simulink model "ASM_Traffic_new"  (R2024a)
settings: Solver=ode1  StartTime=SIM.tstart.v  StopTime=SIM.tend.v  FixedStep=SIM.StepSize.v  RelTol=1e-3
PostLoadFcn:
  | if any(exist('dsrtsu_mdlpostloadfcn', 'file') ~= 0), dsrtsu_mdlpostloadfcn('Execute', bdroot); end
  | try, asm_mdl_postloadfcn(bdroot, 'UpdateModel', 3600); catch, disp(lasterr); end,
InitFcn:
  | , if any(exist('rtifpga_mdlclblib', 'file') ~= 0), rtifpga_mdlclblib('Init', bdroot); end,
  | , if any(exist('dsmpb_private', 'file') ~= 0), dsmpb_private('dsmpb_mdlclblib', 'Init', bdroot); end,
undefined symbols (not defined in the file): _to_, a0b2, ASM_BrakeHydraulics_DemoSystems, ASM_VehicleDynamics_DemoSystems, b98103fe8ad365046cd0, BrakeCircuit, CPT, Crankshaft, DiscIntNeverNeededParam, dsmsi, FinalDriveAssembly, MDL, ModeSignals, Pos_BrakePedal_Maneuver, rad, RefSignals, s_to_rpm, SIM, SoftECU, Suspension, Tire, Transmission
libraries: ASM_Traffic_lib x135, simulink x100, ASM_Utils_lib x77, ASM_VehicleDynamics_lib x70, ASM_Environment_lib x22, dsmpblib x20, dsmsilib x15, MDLD_Utils_lib x10, ASM_BrakeHydraulics_lib x3
(part 52 of 63)

== system ASM_Traffic_new/Environment/Traffic/UserInterface/PAR_Plant/Fellow_Doors/Fellow26_Doors ==
  Bus Creator1 : BusCreator  Inputs=7
  SW_DoorFL[0Closed_1Open] : Constant  Value=0
  SW_DoorFR[0Closed_1Open] : Constant  Value=0
  SW_DoorRL[0Closed_1Open] : Constant  Value=0
  SW_DoorRR[0Closed_1Open] : Constant  Value=0
  SW_Hood[0Closed_1Open] : Constant  Value=0
  SW_ManualControl_Doors[1Scheduler|2Manual] : Constant
  SW_Trunk[0Closed_1Open] : Constant  Value=0
  Out1 : Outport  VectorParamsAs1DForOutWhenUnconnected=off
  wires:
  Bus Creator1/1 -> Out1/1
  SW_ManualControl_Doors[1Scheduler|2Manual]/1 -> Bus Creator1/1  "SW_ManualControl_Doors[1Scheduler|2Manual]"
  SW_DoorFL[0Closed_1Open]/1 -> Bus Creator1/2  "SW_DoorFL[0Closed_1Open]"
  SW_DoorFR[0Closed_1Open]/1 -> Bus Creator1/3  "SW_DoorFR[0Closed_1Open]"
  SW_DoorRL[0Closed_1Open]/1 -> Bus Creator1/4  "SW_DoorRL[0Closed_1Open]"
  SW_DoorRR[0Closed_1Open]/1 -> Bus Creator1/5  "SW_DoorRR[0Closed_1Open]"
  SW_Hood[0Closed_1Open]/1 -> Bus Creator1/6  "SW_Hood[0Closed_1Open]"
  SW_Trunk[0Closed_1Open]/1 -> Bus Creator1/7  "SW_Trunk[0Closed_1Open]"

== system ASM_Traffic_new/Environment/Traffic/UserInterface/PAR_Plant/Fellow_Doors/Fellow27_Doors ==
  Bus Creator1 : BusCreator  Inputs=7
  SW_DoorFL[0Closed_1Open] : Constant  Value=0
  SW_DoorFR[0Closed_1Open] : Constant  Value=0
  SW_DoorRL[0Closed_1Open] : Constant  Value=0
  SW_DoorRR[0Closed_1Open] : Constant  Value=0
  SW_Hood[0Closed_1Open] : Constant  Value=0
  SW_ManualControl_Doors[1Scheduler|2Manual] : Constant
  SW_Trunk[0Closed_1Open] : Constant  Value=0
  Out1 : Outport  VectorParamsAs1DForOutWhenUnconnected=off
  wires:
  Bus Creator1/1 -> Out1/1
  SW_ManualControl_Doors[1Scheduler|2Manual]/1 -> Bus Creator1/1  "SW_ManualControl_Doors[1Scheduler|2Manual]"
  SW_DoorFL[0Closed_1Open]/1 -> Bus Creator1/2  "SW_DoorFL[0Closed_1Open]"
  SW_DoorFR[0Closed_1Open]/1 -> Bus Creator1/3  "SW_DoorFR[0Closed_1Open]"
  SW_DoorRL[0Closed_1Open]/1 -> Bus Creator1/4  "SW_DoorRL[0Closed_1Open]"
  SW_DoorRR[0Closed_1Open]/1 -> Bus Creator1/5  "SW_DoorRR[0Closed_1Open]"
  SW_Hood[0Closed_1Open]/1 -> Bus Creator1/6  "SW_Hood[0Closed_1Open]"
  SW_Trunk[0Closed_1Open]/1 -> Bus Creator1/7  "SW_Trunk[0Closed_1Open]"

== system ASM_Traffic_new/Environment/Traffic/UserInterface/PAR_Plant/Fellow_Doors/Fellow28_Doors ==
  Bus Creator1 : BusCreator  Inputs=7
  SW_DoorFL[0Closed_1Open] : Constant  Value=0
  SW_DoorFR[0Closed_1Open] : Constant  Value=0
  SW_DoorRL[0Closed_1Open] : Constant  Value=0
  SW_DoorRR[0Closed_1Open] : Constant  Value=0
  SW_Hood[0Closed_1Open] : Constant  Value=0
  SW_ManualControl_Doors[1Scheduler|2Manual] : Constant
  SW_Trunk[0Closed_1Open] : Constant  Value=0
  Out1 : Outport  VectorParamsAs1DForOutWhenUnconnected=off
  wires:
  Bus Creator1/1 -> Out1/1
  SW_ManualControl_Doors[1Scheduler|2Manual]/1 -> Bus Creator1/1  "SW_ManualControl_Doors[1Scheduler|2Manual]"
  SW_DoorFL[0Closed_1Open]/1 -> Bus Creator1/2  "SW_DoorFL[0Closed_1Open]"
  SW_DoorFR[0Closed_1Open]/1 -> Bus Creator1/3  "SW_DoorFR[0Closed_1Open]"
  SW_DoorRL[0Closed_1Open]/1 -> Bus Creator1/4  "SW_DoorRL[0Closed_1Open]"
  SW_DoorRR[0Closed_1Open]/1 -> Bus Creator1/5  "SW_DoorRR[0Closed_1Open]"
  SW_Hood[0Closed_1Open]/1 -> Bus Creator1/6  "SW_Hood[0Closed_1Open]"
  SW_Trunk[0Closed_1Open]/1 -> Bus Creator1/7  "SW_Trunk[0Closed_1Open]"

== system ASM_Traffic_new/Environment/Traffic/UserInterface/PAR_Plant/Fellow_Doors/Fellow29_Doors ==
  Bus Creator1 : BusCreator  Inputs=7
  SW_DoorFL[0Closed_1Open] : Constant  Value=0
  SW_DoorFR[0Closed_1Open] : Constant  Value=0
  SW_DoorRL[0Closed_1Open] : Constant  Value=0
  SW_DoorRR[0Closed_1Open] : Constant  Value=0
  SW_Hood[0Closed_1Open] : Constant  Value=0
  SW_ManualControl_Doors[1Scheduler|2Manual] : Constant
  SW_Trunk[0Closed_1Open] : Constant  Value=0
  Out1 : Outport  VectorParamsAs1DForOutWhenUnconnected=off
  wires:
  Bus Creator1/1 -> Out1/1
  SW_ManualControl_Doors[1Scheduler|2Manual]/1 -> Bus Creator1/1  "SW_ManualControl_Doors[1Scheduler|2Manual]"
  SW_DoorFL[0Closed_1Open]/1 -> Bus Creator1/2  "SW_DoorFL[0Closed_1Open]"
  SW_DoorFR[0Closed_1Open]/1 -> Bus Creator1/3  "SW_DoorFR[0Closed_1Open]"
  SW_DoorRL[0Closed_1Open]/1 -> Bus Creator1/4  "SW_DoorRL[0Closed_1Open]"
  SW_DoorRR[0Closed_1Open]/1 -> Bus Creator1/5  "SW_DoorRR[0Closed_1Open]"
  SW_Hood[0Closed_1Open]/1 -> Bus Creator1/6  "SW_Hood[0Closed_1Open]"
  SW_Trunk[0Closed_1Open]/1 -> Bus Creator1/7  "SW_Trunk[0Closed_1Open]"

== system ASM_Traffic_new/Environment/Traffic/UserInterface/PAR_Plant/Fellow_Doors/Fellow2_Doors ==
  Bus Creator1 : BusCreator  Inputs=7
  SW_DoorFL[0Closed_1Open] : Constant  Value=0
  SW_DoorFR[0Closed_1Open] : Constant  Value=0
  SW_DoorRL[0Closed_1Open] : Constant  Value=0
  SW_DoorRR[0Closed_1Open] : Constant  Value=0
  SW_Hood[0Closed_1Open] : Constant  Value=0
  SW_ManualControl_Doors[1Scheduler|2Manual] : Constant
  SW_Trunk[0Closed_1Open] : Constant  Value=0
  Out1 : Outport  VectorParamsAs1DForOutWhenUnconnected=off
  wires:
  Bus Creator1/1 -> Out1/1
  SW_ManualControl_Doors[1Scheduler|2Manual]/1 -> Bus Creator1/1  "SW_ManualControl_Doors[1Scheduler|2Manual]"
  SW_DoorFL[0Closed_1Open]/1 -> Bus Creator1/2  "SW_DoorFL[0Closed_1Open]"
  SW_DoorFR[0Closed_1Open]/1 -> Bus Creator1/3  "SW_DoorFR[0Closed_1Open]"
  SW_DoorRL[0Closed_1Open]/1 -> Bus Creator1/4  "SW_DoorRL[0Closed_1Open]"
  SW_DoorRR[0Closed_1Open]/1 -> Bus Creator1/5  "SW_DoorRR[0Closed_1Open]"
  SW_Hood[0Closed_1Open]/1 -> Bus Creator1/6  "SW_Hood[0Closed_1Open]"
  SW_Trunk[0Closed_1Open]/1 -> Bus Creator1/7  "SW_Trunk[0Closed_1Open]"

== system ASM_Traffic_new/Environment/Traffic/UserInterface/PAR_Plant/Fellow_Doors/Fellow30_Doors ==
  Bus Creator1 : BusCreator  Inputs=7
  SW_DoorFL[0Closed_1Open] : Constant  Value=0
  SW_DoorFR[0Closed_1Open] : Constant  Value=0
  SW_DoorRL[0Closed_1Open] : Constant  Value=0
  SW_DoorRR[0Closed_1Open] : Constant  Value=0
  SW_Hood[0Closed_1Open] : Constant  Value=0
  SW_ManualControl_Doors[1Scheduler|2Manual] : Constant
  SW_Trunk[0Closed_1Open] : Constant  Value=0
  Out1 : Outport  VectorParamsAs1DForOutWhenUnconnected=off
  wires:
  Bus Creator1/1 -> Out1/1
  SW_ManualControl_Doors[1Scheduler|2Manual]/1 -> Bus Creator1/1  "SW_ManualControl_Doors[1Scheduler|2Manual]"
  SW_DoorFL[0Closed_1Open]/1 -> Bus Creator1/2  "SW_DoorFL[0Closed_1Open]"
  SW_DoorFR[0Closed_1Open]/1 -> Bus Creator1/3  "SW_DoorFR[0Closed_1Open]"
  SW_DoorRL[0Closed_1Open]/1 -> Bus Creator1/4  "SW_DoorRL[0Closed_1Open]"
  SW_DoorRR[0Closed_1Open]/1 -> Bus Creator1/5  "SW_DoorRR[0Closed_1Open]"
  SW_Hood[0Closed_1Open]/1 -> Bus Creator1/6  "SW_Hood[0Closed_1Open]"
  SW_Trunk[0Closed_1Open]/1 -> Bus Creator1/7  "SW_Trunk[0Closed_1Open]"

== system ASM_Traffic_new/Environment/Traffic/UserInterface/PAR_Plant/Fellow_Doors/Fellow3_Doors ==
  Bus Creator1 : BusCreator  Inputs=7
  SW_DoorFL[0Closed_1Open] : Constant  Value=0
  SW_DoorFR[0Closed_1Open] : Constant  Value=0
  SW_DoorRL[0Closed_1Open] : Constant  Value=0
  SW_DoorRR[0Closed_1Open] : Constant  Value=0
  SW_Hood[0Closed_1Open] : Constant  Value=0
  SW_ManualControl_Doors[1Scheduler|2Manual] : Constant
  SW_Trunk[0Closed_1Open] : Constant  Value=0
  Out1 : Outport  VectorParamsAs1DForOutWhenUnconnected=off
  wires:
  Bus Creator1/1 -> Out1/1
  SW_ManualControl_Doors[1Scheduler|2Manual]/1 -> Bus Creator1/1  "SW_ManualControl_Doors[1Scheduler|2Manual]"
  SW_DoorFL[0Closed_1Open]/1 -> Bus Creator1/2  "SW_DoorFL[0Closed_1Open]"
  SW_DoorFR[0Closed_1Open]/1 -> Bus Creator1/3  "SW_DoorFR[0Closed_1Open]"
  SW_DoorRL[0Closed_1Open]/1 -> Bus Creator1/4  "SW_DoorRL[0Closed_1Open]"
  SW_DoorRR[0Closed_1Open]/1 -> Bus Creator1/5  "SW_DoorRR[0Closed_1Open]"
  SW_Hood[0Closed_1Open]/1 -> Bus Creator1/6  "SW_Hood[0Closed_1Open]"
  SW_Trunk[0Closed_1Open]/1 -> Bus Creator1/7  "SW_Trunk[0Closed_1Open]"

== system ASM_Traffic_new/Environment/Traffic/UserInterface/PAR_Plant/Fellow_Doors/Fellow4_Doors ==
  Bus Creator1 : BusCreator  Inputs=7
  SW_DoorFL[0Closed_1Open] : Constant  Value=0
  SW_DoorFR[0Closed_1Open] : Constant  Value=0
  SW_DoorRL[0Closed_1Open] : Constant  Value=0
  SW_DoorRR[0Closed_1Open] : Constant  Value=0
  SW_Hood[0Closed_1Open] : Constant  Value=0
  SW_ManualControl_Doors[1Scheduler|2Manual] : Constant
  SW_Trunk[0Closed_1Open] : Constant  Value=0
  Out1 : Outport  VectorParamsAs1DForOutWhenUnconnected=off
  wires:
  Bus Creator1/1 -> Out1/1
  SW_ManualControl_Doors[1Scheduler|2Manual]/1 -> Bus Creator1/1  "SW_ManualControl_Doors[1Scheduler|2Manual]"
  SW_DoorFL[0Closed_1Open]/1 -> Bus Creator1/2  "SW_DoorFL[0Closed_1Open]"
  SW_DoorFR[0Closed_1Open]/1 -> Bus Creator1/3  "SW_DoorFR[0Closed_1Open]"
  SW_DoorRL[0Closed_1Open]/1 -> Bus Creator1/4  "SW_DoorRL[0Closed_1Open]"
  SW_DoorRR[0Closed_1Open]/1 -> Bus Creator1/5  "SW_DoorRR[0Closed_1Open]"
  SW_Hood[0Closed_1Open]/1 -> Bus Creator1/6  "SW_Hood[0Closed_1Open]"
  SW_Trunk[0Closed_1Open]/1 -> Bus Creator1/7  "SW_Trunk[0Closed_1Open]"

== system ASM_Traffic_new/Environment/Traffic/UserInterface/PAR_Plant/Fellow_Doors/Fellow5_Doors ==
  Bus Creator1 : BusCreator  Inputs=7
  SW_DoorFL[0Closed_1Open] : Constant  Value=0
  SW_DoorFR[0Closed_1Open] : Constant  Value=0
  SW_DoorRL[0Closed_1Open] : Constant  Value=0
  SW_DoorRR[0Closed_1Open] : Constant  Value=0
  SW_Hood[0Closed_1Open] : Constant  Value=0
  SW_ManualControl_Doors[1Scheduler|2Manual] : Constant
  SW_Trunk[0Closed_1Open] : Constant  Value=0
  Out1 : Outport  VectorParamsAs1DForOutWhenUnconnected=off
  wires:
  Bus Creator1/1 -> Out1/1
  SW_ManualControl_Doors[1Scheduler|2Manual]/1 -> Bus Creator1/1  "SW_ManualControl_Doors[1Scheduler|2Manual]"
  SW_DoorFL[0Closed_1Open]/1 -> Bus Creator1/2  "SW_DoorFL[0Closed_1Open]"
  SW_DoorFR[0Closed_1Open]/1 -> Bus Creator1/3  "SW_DoorFR[0Closed_1Open]"
  SW_DoorRL[0Closed_1Open]/1 -> Bus Creator1/4  "SW_DoorRL[0Closed_1Open]"
  SW_DoorRR[0Closed_1Open]/1 -> Bus Creator1/5  "SW_DoorRR[0Closed_1Open]"
  SW_Hood[0Closed_1Open]/1 -> Bus Creator1/6  "SW_Hood[0Closed_1Open]"
  SW_Trunk[0Closed_1Open]/1 -> Bus Creator1/7  "SW_Trunk[0Closed_1Open]"

== system ASM_Traffic_new/Environment/Traffic/UserInterface/PAR_Plant/Fellow_Doors/Fellow6_Doors ==
  Bus Creator1 : BusCreator  Inputs=7
  SW_DoorFL[0Closed_1Open] : Constant  Value=0
  SW_DoorFR[0Closed_1Open] : Constant  Value=0
  SW_DoorRL[0Closed_1Open] : Constant  Value=0
  SW_DoorRR[0Closed_1Open] : Constant  Value=0
  SW_Hood[0Closed_1Open] : Constant  Value=0
  SW_ManualControl_Doors[1Scheduler|2Manual] : Constant
  SW_Trunk[0Closed_1Open] : Constant  Value=0
  Out1 : Outport  VectorParamsAs1DForOutWhenUnconnected=off
  wires:
  Bus Creator1/1 -> Out1/1
  SW_ManualControl_Doors[1Scheduler|2Manual]/1 -> Bus Creator1/1  "SW_ManualControl_Doors[1Scheduler|2Manual]"
  SW_DoorFL[0Closed_1Open]/1 -> Bus Creator1/2  "SW_DoorFL[0Closed_1Open]"
  SW_DoorFR[0Closed_1Open]/1 -> Bus Creator1/3  "SW_DoorFR[0Closed_1Open]"
  SW_DoorRL[0Closed_1Open]/1 -> Bus Creator1/4  "SW_DoorRL[0Closed_1Open]"
  SW_DoorRR[0Closed_1Open]/1 -> Bus Creator1/5  "SW_DoorRR[0Closed_1Open]"
  SW_Hood[0Closed_1Open]/1 -> Bus Creator1/6  "SW_Hood[0Closed_1Open]"
  SW_Trunk[0Closed_1Open]/1 -> Bus Creator1/7  "SW_Trunk[0Closed_1Open]"

== system ASM_Traffic_new/Environment/Traffic/UserInterface/PAR_Plant/Fellow_Doors/Fellow7_Doors ==
  Bus Creator1 : BusCreator  Inputs=7
  SW_DoorFL[0Closed_1Open] : Constant  Value=0
  SW_DoorFR[0Closed_1Open] : Constant  Value=0
  SW_DoorRL[0Closed_1Open] : Constant  Value=0
  SW_DoorRR[0Closed_1Open] : Constant  Value=0
  SW_Hood[0Closed_1Open] : Constant  Value=0
  SW_ManualControl_Doors[1Scheduler|2Manual] : Constant
  SW_Trunk[0Closed_1Open] : Constant  Value=0
  Out1 : Outport  VectorParamsAs1DForOutWhenUnconnected=off
  wires:
  Bus Creator1/1 -> Out1/1
  SW_ManualControl_Doors[1Scheduler|2Manual]/1 -> Bus Creator1/1  "SW_ManualControl_Doors[1Scheduler|2Manual]"
  SW_DoorFL[0Closed_1Open]/1 -> Bus Creator1/2  "SW_DoorFL[0Closed_1Open]"
  SW_DoorFR[0Closed_1Open]/1 -> Bus Creator1/3  "SW_DoorFR[0Closed_1Open]"
  SW_DoorRL[0Closed_1Open]/1 -> Bus Creator1/4  "SW_DoorRL[0Closed_1Open]"
  SW_DoorRR[0Closed_1Open]/1 -> Bus Creator1/5  "SW_DoorRR[0Closed_1Open]"
  SW_Hood[0Closed_1Open]/1 -> Bus Creator1/6  "SW_Hood[0Closed_1Open]"
  SW_Trunk[0Closed_1Open]/1 -> Bus Creator1/7  "SW_Trunk[0Closed_1Open]"

== system ASM_Traffic_new/Environment/Traffic/UserInterface/PAR_Plant/Fellow_Doors/Fellow8_Doors ==
  Bus Creator1 : BusCreator  Inputs=7
  SW_DoorFL[0Closed_1Open] : Constant  Value=0
  SW_DoorFR[0Closed_1Open] : Constant  Value=0
  SW_DoorRL[0Closed_1Open] : Constant  Value=0
  SW_DoorRR[0Closed_1Open] : Constant  Value=0
  SW_Hood[0Closed_1Open] : Constant  Value=0
  SW_ManualControl_Doors[1Scheduler|2Manual] : Constant
  SW_Trunk[0Closed_1Open] : Constant  Value=0
  Out1 : Outport  VectorParamsAs1DForOutWhenUnconnected=off
  wires:
  Bus Creator1/1 -> Out1/1
  SW_ManualControl_Doors[1Scheduler|2Manual]/1 -> Bus Creator1/1  "SW_ManualControl_Doors[1Scheduler|2Manual]"
  SW_DoorFL[0Closed_1Open]/1 -> Bus Creator1/2  "SW_DoorFL[0Closed_1Open]"
  SW_DoorFR[0Closed_1Open]/1 -> Bus Creator1/3  "SW_DoorFR[0Closed_1Open]"
  SW_DoorRL[0Closed_1Open]/1 -> Bus Creator1/4  "SW_DoorRL[0Closed_1Open]"
  SW_DoorRR[0Closed_1Open]/1 -> Bus Creator1/5  "SW_DoorRR[0Closed_1Open]"
  SW_Hood[0Closed_1Open]/1 -> Bus Creator1/6  "SW_Hood[0Closed_1Open]"
  SW_Trunk[0Closed_1Open]/1 -> Bus Creator1/7  "SW_Trunk[0Closed_1Open]"

== system ASM_Traffic_new/Environment/Traffic/UserInterface/PAR_Plant/Fellow_Doors/Fellow9_Doors ==
  Bus Creator1 : BusCreator  Inputs=7
  SW_DoorFL[0Closed_1Open] : Constant  Value=0
  SW_DoorFR[0Closed_1Open] : Constant  Value=0
  SW_DoorRL[0Closed_1Open] : Constant  Value=0
  SW_DoorRR[0Closed_1Open] : Constant  Value=0
  SW_Hood[0Closed_1Open] : Constant  Value=0
  SW_ManualControl_Doors[1Scheduler|2Manual] : Constant
  SW_Trunk[0Closed_1Open] : Constant  Value=0
  Out1 : Outport  VectorParamsAs1DForOutWhenUnconnected=off
  wires:
  Bus Creator1/1 -> Out1/1
  SW_ManualControl_Doors[1Scheduler|2Manual]/1 -> Bus Creator1/1  "SW_ManualControl_Doors[1Scheduler|2Manual]"
  SW_DoorFL[0Closed_1Open]/1 -> Bus Creator1/2  "SW_DoorFL[0Closed_1Open]"
  SW_DoorFR[0Closed_1Open]/1 -> Bus Creator1/3  "SW_DoorFR[0Closed_1Open]"
  SW_DoorRL[0Closed_1Open]/1 -> Bus Creator1/4  "SW_DoorRL[0Closed_1Open]"
  SW_DoorRR[0Closed_1Open]/1 -> Bus Creator1/5  "SW_DoorRR[0Closed_1Open]"
  SW_Hood[0Closed_1Open]/1 -> Bus Creator1/6  "SW_Hood[0Closed_1Open]"
  SW_Trunk[0Closed_1Open]/1 -> Bus Creator1/7  "SW_Trunk[0Closed_1Open]"

== system ASM_Traffic_new/Environment/Traffic/UserInterface/PAR_Plant/Fellow_VehicleLights/Fellow10_VehicleLights ==
  Bus Creator1 : BusCreator  Inputs=3
  SW_BrakeLight[0Off|1On] : Constant  Value=0
  SW_ManualControl_Lights[1Scheduler|2Manual] : Constant
  SW_TurnLights[0Off|1Left|2Right|3Both] : Constant  Value=0
  Out1 : Outport  VectorParamsAs1DForOutWhenUnconnected=off
  wires:
  SW_ManualControl_Lights[1Scheduler|2Manual]/1 -> Bus Creator1/1  "SW_ManualControl_Lights[1Scheduler|2Manual]"
  SW_TurnLights[0Off|1Left|2Right|3Both]/1 -> Bus Creator1/3  "SW_TurnLights[0Off|1Left|2Right|3Both]"
  SW_BrakeLight[0Off|1On]/1 -> Bus Creator1/2  "SW_BrakeLight[0Off|1On]"
  Bus Creator1/1 -> Out1/1

== system ASM_Traffic_new/Environment/Traffic/UserInterface/PAR_Plant/Fellow_VehicleLights/Fellow11_VehicleLights ==
  Bus Creator1 : BusCreator  Inputs=3
  SW_BrakeLight[0Off|1On] : Constant  Value=0
  SW_ManualControl_Lights[1Scheduler|2Manual] : Constant
  SW_TurnLights[0Off|1Left|2Right|3Both] : Constant  Value=0
  Out1 : Outport  VectorParamsAs1DForOutWhenUnconnected=off
  wires:
  Bus Creator1/1 -> Out1/1
  SW_BrakeLight[0Off|1On]/1 -> Bus Creator1/2  "SW_BrakeLight[0Off|1On]"
  SW_TurnLights[0Off|1Left|2Right|3Both]/1 -> Bus Creator1/3  "SW_TurnLights[0Off|1Left|2Right|3Both]"
  SW_ManualControl_Lights[1Scheduler|2Manual]/1 -> Bus Creator1/1  "SW_ManualControl_Lights[1Scheduler|2Manual]"

== system ASM_Traffic_new/Environment/Traffic/UserInterface/PAR_Plant/Fellow_VehicleLights/Fellow12_VehicleLights ==
  Bus Creator1 : BusCreator  Inputs=3
  SW_BrakeLight[0Off|1On] : Constant  Value=0
  SW_ManualControl_Lights[1Scheduler|2Manual] : Constant
  SW_TurnLights[0Off|1Left|2Right|3Both] : Constant  Value=0
  Out1 : Outport  VectorParamsAs1DForOutWhenUnconnected=off
  wires:
  SW_ManualControl_Lights[1Scheduler|2Manual]/1 -> Bus Creator1/1  "SW_ManualControl_Lights[1Scheduler|2Manual]"
  SW_TurnLights[0Off|1Left|2Right|3Both]/1 -> Bus Creator1/3  "SW_TurnLights[0Off|1Left|2Right|3Both]"
  SW_BrakeLight[0Off|1On]/1 -> Bus Creator1/2  "SW_BrakeLight[0Off|1On]"
  Bus Creator1/1 -> Out1/1

== system ASM_Traffic_new/Environment/Traffic/UserInterface/PAR_Plant/Fellow_VehicleLights/Fellow13_VehicleLights ==
  Bus Creator1 : BusCreator  Inputs=3
  SW_BrakeLight[0Off|1On] : Constant  Value=0
  SW_ManualControl_Lights[1Scheduler|2Manual] : Constant
  SW_TurnLights[0Off|1Left|2Right|3Both] : Constant  Value=0
  Out1 : Outport  VectorParamsAs1DForOutWhenUnconnected=off
  wires:
  Bus Creator1/1 -> Out1/1
  SW_BrakeLight[0Off|1On]/1 -> Bus Creator1/2  "SW_BrakeLight[0Off|1On]"
  SW_TurnLights[0Off|1Left|2Right|3Both]/1 -> Bus Creator1/3  "SW_TurnLights[0Off|1Left|2Right|3Both]"
  SW_ManualControl_Lights[1Scheduler|2Manual]/1 -> Bus Creator1/1  "SW_ManualControl_Lights[1Scheduler|2Manual]"

== system ASM_Traffic_new/Environment/Traffic/UserInterface/PAR_Plant/Fellow_VehicleLights/Fellow14_VehicleLights ==
  Bus Creator1 : BusCreator  Inputs=3
  SW_BrakeLight[0Off|1On] : Constant  Value=0
  SW_ManualControl_Lights[1Scheduler|2Manual] : Constant
  SW_TurnLights[0Off|1Left|2Right|3Both] : Constant  Value=0
  Out1 : Outport  VectorParamsAs1DForOutWhenUnconnected=off
  wires:
  SW_ManualControl_Lights[1Scheduler|2Manual]/1 -> Bus Creator1/1  "SW_ManualControl_Lights[1Scheduler|2Manual]"
  SW_TurnLights[0Off|1Left|2Right|3Both]/1 -> Bus Creator1/3  "SW_TurnLights[0Off|1Left|2Right|3Both]"
  SW_BrakeLight[0Off|1On]/1 -> Bus Creator1/2  "SW_BrakeLight[0Off|1On]"
  Bus Creator1/1 -> Out1/1

== system ASM_Traffic_new/Environment/Traffic/UserInterface/PAR_Plant/Fellow_VehicleLights/Fellow15_VehicleLights ==
  Bus Creator1 : BusCreator  Inputs=3
  SW_BrakeLight[0Off|1On] : Constant  Value=0
  SW_ManualControl_Lights[1Scheduler|2Manual] : Constant
  SW_TurnLights[0Off|1Left|2Right|3Both] : Constant  Value=0
  Out1 : Outport  VectorParamsAs1DForOutWhenUnconnected=off
  wires:
  Bus Creator1/1 -> Out1/1
  SW_BrakeLight[0Off|1On]/1 -> Bus Creator1/2  "SW_BrakeLight[0Off|1On]"
  SW_TurnLights[0Off|1Left|2Right|3Both]/1 -> Bus Creator1/3  "SW_TurnLights[0Off|1Left|2Right|3Both]"
  SW_ManualControl_Lights[1Scheduler|2Manual]/1 -> Bus Creator1/1  "SW_ManualControl_Lights[1Scheduler|2Manual]"

== system ASM_Traffic_new/Environment/Traffic/UserInterface/PAR_Plant/Fellow_VehicleLights/Fellow16_VehicleLights ==
  Bus Creator1 : BusCreator  Inputs=3
  SW_BrakeLight[0Off|1On] : Constant  Value=0
  SW_ManualControl_Lights[1Scheduler|2Manual] : Constant
  SW_TurnLights[0Off|1Left|2Right|3Both] : Constant  Value=0
  Out1 : Outport  VectorParamsAs1DForOutWhenUnconnected=off
  wires:
  SW_ManualControl_Lights[1Scheduler|2Manual]/1 -> Bus Creator1/1  "SW_ManualControl_Lights[1Scheduler|2Manual]"
  SW_TurnLights[0Off|1Left|2Right|3Both]/1 -> Bus Creator1/3  "SW_TurnLights[0Off|1Left|2Right|3Both]"
  SW_BrakeLight[0Off|1On]/1 -> Bus Creator1/2  "SW_BrakeLight[0Off|1On]"
  Bus Creator1/1 -> Out1/1

== system ASM_Traffic_new/Environment/Traffic/UserInterface/PAR_Plant/Fellow_VehicleLights/Fellow17_VehicleLights ==
  Bus Creator1 : BusCreator  Inputs=3
  SW_BrakeLight[0Off|1On] : Constant  Value=0
  SW_ManualControl_Lights[1Scheduler|2Manual] : Constant
  SW_TurnLights[0Off|1Left|2Right|3Both] : Constant  Value=0
  Out1 : Outport  VectorParamsAs1DForOutWhenUnconnected=off
  wires:
  Bus Creator1/1 -> Out1/1
  SW_BrakeLight[0Off|1On]/1 -> Bus Creator1/2  "SW_BrakeLight[0Off|1On]"
  SW_TurnLights[0Off|1Left|2Right|3Both]/1 -> Bus Creator1/3  "SW_TurnLights[0Off|1Left|2Right|3Both]"
  SW_ManualControl_Lights[1Scheduler|2Manual]/1 -> Bus Creator1/1  "SW_ManualControl_Lights[1Scheduler|2Manual]"

== system ASM_Traffic_new/Environment/Traffic/UserInterface/PAR_Plant/Fellow_VehicleLights/Fellow18_VehicleLights ==
  Bus Creator1 : BusCreator  Inputs=3
  SW_BrakeLight[0Off|1On] : Constant  Value=0
  SW_ManualControl_Lights[1Scheduler|2Manual] : Constant
  SW_TurnLights[0Off|1Left|2Right|3Both] : Constant  Value=0
  Out1 : Outport  VectorParamsAs1DForOutWhenUnconnected=off
  wires:
  SW_ManualControl_Lights[1Scheduler|2Manual]/1 -> Bus Creator1/1  "SW_ManualControl_Lights[1Scheduler|2Manual]"
  SW_TurnLights[0Off|1Left|2Right|3Both]/1 -> Bus Creator1/3  "SW_TurnLights[0Off|1Left|2Right|3Both]"
  SW_BrakeLight[0Off|1On]/1 -> Bus Creator1/2  "SW_BrakeLight[0Off|1On]"
  Bus Creator1/1 -> Out1/1

== system ASM_Traffic_new/Environment/Traffic/UserInterface/PAR_Plant/Fellow_VehicleLights/Fellow19_VehicleLights ==
  Bus Creator1 : BusCreator  Inputs=3
  SW_BrakeLight[0Off|1On] : Constant  Value=0
  SW_ManualControl_Lights[1Scheduler|2Manual] : Constant
  SW_TurnLights[0Off|1Left|2Right|3Both] : Constant  Value=0
  Out1 : Outport  VectorParamsAs1DForOutWhenUnconnected=off
  wires:
  Bus Creator1/1 -> Out1/1
  SW_BrakeLight[0Off|1On]/1 -> Bus Creator1/2  "SW_BrakeLight[0Off|1On]"
  SW_TurnLights[0Off|1Left|2Right|3Both]/1 -> Bus Creator1/3  "SW_TurnLights[0Off|1Left|2Right|3Both]"
  SW_ManualControl_Lights[1Scheduler|2Manual]/1 -> Bus Creator1/1  "SW_ManualControl_Lights[1Scheduler|2Manual]"

== system ASM_Traffic_new/Environment/Traffic/UserInterface/PAR_Plant/Fellow_VehicleLights/Fellow1_VehicleLights ==
  Bus Creator1 : BusCreator  Inputs=3
  SW_BrakeLight[0Off|1On] : Constant  Value=0
  SW_ManualControl_Lights[1Scheduler|2Manual] : Constant
  SW_TurnLights[0Off|1Left|2Right|3Both] : Constant  Value=0
  Out1 : Outport  VectorParamsAs1DForOutWhenUnconnected=off
  wires:
  Bus Creator1/1 -> Out1/1
  SW_BrakeLight[0Off|1On]/1 -> Bus Creator1/2  "SW_BrakeLight[0Off|1On]"
  SW_TurnLights[0Off|1Left|2Right|3Both]/1 -> Bus Creator1/3  "SW_TurnLights[0Off|1Left|2Right|3Both]"
  SW_ManualControl_Lights[1Scheduler|2Manual]/1 -> Bus Creator1/1  "SW_ManualControl_Lights[1Scheduler|2Manual]"

== system ASM_Traffic_new/Environment/Traffic/UserInterface/PAR_Plant/Fellow_VehicleLights/Fellow20_VehicleLights ==
  Bus Creator1 : BusCreator  Inputs=3
  SW_BrakeLight[0Off|1On] : Constant  Value=0
  SW_ManualControl_Lights[1Scheduler|2Manual] : Constant
  SW_TurnLights[0Off|1Left|2Right|3Both] : Constant  Value=0
  Out1 : Outport  VectorParamsAs1DForOutWhenUnconnected=off
  wires:
  SW_ManualControl_Lights[1Scheduler|2Manual]/1 -> Bus Creator1/1  "SW_ManualControl_Lights[1Scheduler|2Manual]"
  SW_TurnLights[0Off|1Left|2Right|3Both]/1 -> Bus Creator1/3  "SW_TurnLights[0Off|1Left|2Right|3Both]"
  SW_BrakeLight[0Off|1On]/1 -> Bus Creator1/2  "SW_BrakeLight[0Off|1On]"
  Bus Creator1/1 -> Out1/1

== system ASM_Traffic_new/Environment/Traffic/UserInterface/PAR_Plant/Fellow_VehicleLights/Fellow21_VehicleLights ==
  Bus Creator1 : BusCreator  Inputs=3
  SW_BrakeLight[0Off|1On] : Constant  Value=0
  SW_ManualControl_Lights[1Scheduler|2Manual] : Constant
  SW_TurnLights[0Off|1Left|2Right|3Both] : Constant  Value=0
  Out1 : Outport  VectorParamsAs1DForOutWhenUnconnected=off
  wires:
  Bus Creator1/1 -> Out1/1
  SW_BrakeLight[0Off|1On]/1 -> Bus Creator1/2  "SW_BrakeLight[0Off|1On]"
  SW_TurnLights[0Off|1Left|2Right|3Both]/1 -> Bus Creator1/3  "SW_TurnLights[0Off|1Left|2Right|3Both]"
  SW_ManualControl_Lights[1Scheduler|2Manual]/1 -> Bus Creator1/1  "SW_ManualControl_Lights[1Scheduler|2Manual]"

== system ASM_Traffic_new/Environment/Traffic/UserInterface/PAR_Plant/Fellow_VehicleLights/Fellow22_VehicleLights ==
  Bus Creator1 : BusCreator  Inputs=3
  SW_BrakeLight[0Off|1On] : Constant  Value=0
  SW_ManualControl_Lights[1Scheduler|2Manual] : Constant
  SW_TurnLights[0Off|1Left|2Right|3Both] : Constant  Value=0
  Out1 : Outport  VectorParamsAs1DForOutWhenUnconnected=off
  wires:
  SW_ManualControl_Lights[1Scheduler|2Manual]/1 -> Bus Creator1/1  "SW_ManualControl_Lights[1Scheduler|2Manual]"
  SW_TurnLights[0Off|1Left|2Right|3Both]/1 -> Bus Creator1/3  "SW_TurnLights[0Off|1Left|2Right|3Both]"
  SW_BrakeLight[0Off|1On]/1 -> Bus Creator1/2  "SW_BrakeLight[0Off|1On]"
  Bus Creator1/1 -> Out1/1

== system ASM_Traffic_new/Environment/Traffic/UserInterface/PAR_Plant/Fellow_VehicleLights/Fellow23_VehicleLights ==
  Bus Creator1 : BusCreator  Inputs=3
  SW_BrakeLight[0Off|1On] : Constant  Value=0
  SW_ManualControl_Lights[1Scheduler|2Manual] : Constant
  SW_TurnLights[0Off|1Left|2Right|3Both] : Constant  Value=0
  Out1 : Outport  VectorParamsAs1DForOutWhenUnconnected=off
  wires:
  Bus Creator1/1 -> Out1/1
  SW_BrakeLight[0Off|1On]/1 -> Bus Creator1/2  "SW_BrakeLight[0Off|1On]"
  SW_TurnLights[0Off|1Left|2Right|3Both]/1 -> Bus Creator1/3  "SW_TurnLights[0Off|1Left|2Right|3Both]"
  SW_ManualControl_Lights[1Scheduler|2Manual]/1 -> Bus Creator1/1  "SW_ManualControl_Lights[1Scheduler|2Manual]"

== system ASM_Traffic_new/Environment/Traffic/UserInterface/PAR_Plant/Fellow_VehicleLights/Fellow24_VehicleLights ==
  Bus Creator1 : BusCreator  Inputs=3
  SW_BrakeLight[0Off|1On] : Constant  Value=0
  SW_ManualControl_Lights[1Scheduler|2Manual] : Constant
  SW_TurnLights[0Off|1Left|2Right|3Both] : Constant  Value=0
  Out1 : Outport  VectorParamsAs1DForOutWhenUnconnected=off
  wires:
  SW_ManualControl_Lights[1Scheduler|2Manual]/1 -> Bus Creator1/1  "SW_ManualControl_Lights[1Scheduler|2Manual]"
  SW_TurnLights[0Off|1Left|2Right|3Both]/1 -> Bus Creator1/3  "SW_TurnLights[0Off|1Left|2Right|3Both]"
  SW_BrakeLight[0Off|1On]/1 -> Bus Creator1/2  "SW_BrakeLight[0Off|1On]"
  Bus Creator1/1 -> Out1/1

== system ASM_Traffic_new/Environment/Traffic/UserInterface/PAR_Plant/Fellow_VehicleLights/Fellow25_VehicleLights ==
  Bus Creator1 : BusCreator  Inputs=3
  SW_BrakeLight[0Off|1On] : Constant  Value=0
  SW_ManualControl_Lights[1Scheduler|2Manual] : Constant
  SW_TurnLights[0Off|1Left|2Right|3Both] : Constant  Value=0
  Out1 : Outport  VectorParamsAs1DForOutWhenUnconnected=off
  wires:
  Bus Creator1/1 -> Out1/1
  SW_BrakeLight[0Off|1On]/1 -> Bus Creator1/2  "SW_BrakeLight[0Off|1On]"
  SW_TurnLights[0Off|1Left|2Right|3Both]/1 -> Bus Creator1/3  "SW_TurnLights[0Off|1Left|2Right|3Both]"
  SW_ManualControl_Lights[1Scheduler|2Manual]/1 -> Bus Creator1/1  "SW_ManualControl_Lights[1Scheduler|2Manual]"

== system ASM_Traffic_new/Environment/Traffic/UserInterface/PAR_Plant/Fellow_VehicleLights/Fellow26_VehicleLights ==
  Bus Creator1 : BusCreator  Inputs=3
  SW_BrakeLight[0Off|1On] : Constant  Value=0
  SW_ManualControl_Lights[1Scheduler|2Manual] : Constant
  SW_TurnLights[0Off|1Left|2Right|3Both] : Constant  Value=0
  Out1 : Outport  VectorParamsAs1DForOutWhenUnconnected=off
  wires:
  SW_ManualControl_Lights[1Scheduler|2Manual]/1 -> Bus Creator1/1  "SW_ManualControl_Lights[1Scheduler|2Manual]"
  SW_TurnLights[0Off|1Left|2Right|3Both]/1 -> Bus Creator1/3  "SW_TurnLights[0Off|1Left|2Right|3Both]"
  SW_BrakeLight[0Off|1On]/1 -> Bus Creator1/2  "SW_BrakeLight[0Off|1On]"
  Bus Creator1/1 -> Out1/1

== system ASM_Traffic_new/Environment/Traffic/UserInterface/PAR_Plant/Fellow_VehicleLights/Fellow27_VehicleLights ==
  Bus Creator1 : BusCreator  Inputs=3
  SW_BrakeLight[0Off|1On] : Constant  Value=0
  SW_ManualControl_Lights[1Scheduler|2Manual] : Constant
  SW_TurnLights[0Off|1Left|2Right|3Both] : Constant  Value=0
  Out1 : Outport  VectorParamsAs1DForOutWhenUnconnected=off
  wires:
  Bus Creator1/1 -> Out1/1
  SW_BrakeLight[0Off|1On]/1 -> Bus Creator1/2  "SW_BrakeLight[0Off|1On]"
  SW_TurnLights[0Off|1Left|2Right|3Both]/1 -> Bus Creator1/3  "SW_TurnLights[0Off|1Left|2Right|3Both]"
  SW_ManualControl_Lights[1Scheduler|2Manual]/1 -> Bus Creator1/1  "SW_ManualControl_Lights[1Scheduler|2Manual]"

== system ASM_Traffic_new/Environment/Traffic/UserInterface/PAR_Plant/Fellow_VehicleLights/Fellow28_VehicleLights ==
  Bus Creator1 : BusCreator  Inputs=3
  SW_BrakeLight[0Off|1On] : Constant  Value=0
  SW_ManualControl_Lights[1Scheduler|2Manual] : Constant
  SW_TurnLights[0Off|1Left|2Right|3Both] : Constant  Value=0
  Out1 : Outport  VectorParamsAs1DForOutWhenUnconnected=off
  wires:
  SW_ManualControl_Lights[1Scheduler|2Manual]/1 -> Bus Creator1/1  "SW_ManualControl_Lights[1Scheduler|2Manual]"
  SW_TurnLights[0Off|1Left|2Right|3Both]/1 -> Bus Creator1/3  "SW_TurnLights[0Off|1Left|2Right|3Both]"
  SW_BrakeLight[0Off|1On]/1 -> Bus Creator1/2  "SW_BrakeLight[0Off|1On]"
  Bus Creator1/1 -> Out1/1

== system ASM_Traffic_new/Environment/Traffic/UserInterface/PAR_Plant/Fellow_VehicleLights/Fellow29_VehicleLights ==
  Bus Creator1 : BusCreator  Inputs=3
  SW_BrakeLight[0Off|1On] : Constant  Value=0
  SW_ManualControl_Lights[1Scheduler|2Manual] : Constant
  SW_TurnLights[0Off|1Left|2Right|3Both] : Constant  Value=0
  Out1 : Outport  VectorParamsAs1DForOutWhenUnconnected=off
  wires:
  Bus Creator1/1 -> Out1/1
  SW_BrakeLight[0Off|1On]/1 -> Bus Creator1/2  "SW_BrakeLight[0Off|1On]"
  SW_TurnLights[0Off|1Left|2Right|3Both]/1 -> Bus Creator1/3  "SW_TurnLights[0Off|1Left|2Right|3Both]"
  SW_ManualControl_Lights[1Scheduler|2Manual]/1 -> Bus Creator1/1  "SW_ManualControl_Lights[1Scheduler|2Manual]"

== system ASM_Traffic_new/Environment/Traffic/UserInterface/PAR_Plant/Fellow_VehicleLights/Fellow2_VehicleLights ==
  Bus Creator1 : BusCreator  Inputs=3
  SW_BrakeLight[0Off|1On] : Constant  Value=0
  SW_ManualControl_Lights[1Scheduler|2Manual] : Constant
  SW_TurnLights[0Off|1Left|2Right|3Both] : Constant  Value=0
  Out1 : Outport  VectorParamsAs1DForOutWhenUnconnected=off
  wires:
  SW_ManualControl_Lights[1Scheduler|2Manual]/1 -> Bus Creator1/1  "SW_ManualControl_Lights[1Scheduler|2Manual]"
  SW_TurnLights[0Off|1Left|2Right|3Both]/1 -> Bus Creator1/3  "SW_TurnLights[0Off|1Left|2Right|3Both]"
  SW_BrakeLight[0Off|1On]/1 -> Bus Creator1/2  "SW_BrakeLight[0Off|1On]"
  Bus Creator1/1 -> Out1/1

== system ASM_Traffic_new/Environment/Traffic/UserInterface/PAR_Plant/Fellow_VehicleLights/Fellow30_VehicleLights ==
  Bus Creator1 : BusCreator  Inputs=3
  SW_BrakeLight[0Off|1On] : Constant  Value=0
  SW_ManualControl_Lights[1Scheduler|2Manual] : Constant
  SW_TurnLights[0Off|1Left|2Right|3Both] : Constant  Value=0
  Out1 : Outport  VectorParamsAs1DForOutWhenUnconnected=off
  wires:
  SW_ManualControl_Lights[1Scheduler|2Manual]/1 -> Bus Creator1/1  "SW_ManualControl_Lights[1Scheduler|2Manual]"
  SW_TurnLights[0Off|1Left|2Right|3Both]/1 -> Bus Creator1/3  "SW_TurnLights[0Off|1Left|2Right|3Both]"
  SW_BrakeLight[0Off|1On]/1 -> Bus Creator1/2  "SW_BrakeLight[0Off|1On]"
  Bus Creator1/1 -> Out1/1

== system ASM_Traffic_new/Environment/Traffic/UserInterface/PAR_Plant/Fellow_VehicleLights/Fellow3_VehicleLights ==
  Bus Creator1 : BusCreator  Inputs=3
  SW_BrakeLight[0Off|1On] : Constant  Value=0
  SW_ManualControl_Lights[1Scheduler|2Manual] : Constant
  SW_TurnLights[0Off|1Left|2Right|3Both] : Constant  Value=0
  Out1 : Outport  VectorParamsAs1DForOutWhenUnconnected=off
  wires:
  Bus Creator1/1 -> Out1/1
  SW_BrakeLight[0Off|1On]/1 -> Bus Creator1/2  "SW_BrakeLight[0Off|1On]"
  SW_TurnLights[0Off|1Left|2Right|3Both]/1 -> Bus Creator1/3  "SW_TurnLights[0Off|1Left|2Right|3Both]"
  SW_ManualControl_Lights[1Scheduler|2Manual]/1 -> Bus Creator1/1  "SW_ManualControl_Lights[1Scheduler|2Manual]"

== system ASM_Traffic_new/Environment/Traffic/UserInterface/PAR_Plant/Fellow_VehicleLights/Fellow4_VehicleLights ==
  Bus Creator1 : BusCreator  Inputs=3
  SW_BrakeLight[0Off|1On] : Constant  Value=0
  SW_ManualControl_Lights[1Scheduler|2Manual] : Constant
  SW_TurnLights[0Off|1Left|2Right|3Both] : Constant  Value=0
  Out1 : Outport  VectorParamsAs1DForOutWhenUnconnected=off
  wires:
  SW_ManualControl_Lights[1Scheduler|2Manual]/1 -> Bus Creator1/1  "SW_ManualControl_Lights[1Scheduler|2Manual]"
  SW_TurnLights[0Off|1Left|2Right|3Both]/1 -> Bus Creator1/3  "SW_TurnLights[0Off|1Left|2Right|3Both]"
  SW_BrakeLight[0Off|1On]/1 -> Bus Creator1/2  "SW_BrakeLight[0Off|1On]"
  Bus Creator1/1 -> Out1/1

== system ASM_Traffic_new/Environment/Traffic/UserInterface/PAR_Plant/Fellow_VehicleLights/Fellow5_VehicleLights ==
  Bus Creator1 : BusCreator  Inputs=3
  SW_BrakeLight[0Off|1On] : Constant  Value=0
  SW_ManualControl_Lights[1Scheduler|2Manual] : Constant
  SW_TurnLights[0Off|1Left|2Right|3Both] : Constant  Value=0
  Out1 : Outport  VectorParamsAs1DForOutWhenUnconnected=off
  wires:
  Bus Creator1/1 -> Out1/1
  SW_BrakeLight[0Off|1On]/1 -> Bus Creator1/2  "SW_BrakeLight[0Off|1On]"
  SW_TurnLights[0Off|1Left|2Right|3Both]/1 -> Bus Creator1/3  "SW_TurnLights[0Off|1Left|2Right|3Both]"
  SW_ManualControl_Lights[1Scheduler|2Manual]/1 -> Bus Creator1/1  "SW_ManualControl_Lights[1Scheduler|2Manual]"

== system ASM_Traffic_new/Environment/Traffic/UserInterface/PAR_Plant/Fellow_VehicleLights/Fellow6_VehicleLights ==
  Bus Creator1 : BusCreator  Inputs=3
  SW_BrakeLight[0Off|1On] : Constant  Value=0
  SW_ManualControl_Lights[1Scheduler|2Manual] : Constant
  SW_TurnLights[0Off|1Left|2Right|3Both] : Constant  Value=0
  Out1 : Outport  VectorParamsAs1DForOutWhenUnconnected=off
  wires:
  SW_ManualControl_Lights[1Scheduler|2Manual]/1 -> Bus Creator1/1  "SW_ManualControl_Lights[1Scheduler|2Manual]"
  SW_TurnLights[0Off|1Left|2Right|3Both]/1 -> Bus Creator1/3  "SW_TurnLights[0Off|1Left|2Right|3Both]"
  SW_BrakeLight[0Off|1On]/1 -> Bus Creator1/2  "SW_BrakeLight[0Off|1On]"
  Bus Creator1/1 -> Out1/1

== system ASM_Traffic_new/Environment/Traffic/UserInterface/PAR_Plant/Fellow_VehicleLights/Fellow7_VehicleLights ==
  Bus Creator1 : BusCreator  Inputs=3
  SW_BrakeLight[0Off|1On] : Constant  Value=0
  SW_ManualControl_Lights[1Scheduler|2Manual] : Constant
  SW_TurnLights[0Off|1Left|2Right|3Both] : Constant  Value=0
  Out1 : Outport  VectorParamsAs1DForOutWhenUnconnected=off
  wires:
  Bus Creator1/1 -> Out1/1
  SW_BrakeLight[0Off|1On]/1 -> Bus Creator1/2  "SW_BrakeLight[0Off|1On]"
  SW_TurnLights[0Off|1Left|2Right|3Both]/1 -> Bus Creator1/3  "SW_TurnLights[0Off|1Left|2Right|3Both]"
  SW_ManualControl_Lights[1Scheduler|2Manual]/1 -> Bus Creator1/1  "SW_ManualControl_Lights[1Scheduler|2Manual]"

== system ASM_Traffic_new/Environment/Traffic/UserInterface/PAR_Plant/Fellow_VehicleLights/Fellow8_VehicleLights ==
  Bus Creator1 : BusCreator  Inputs=3
  SW_BrakeLight[0Off|1On] : Constant  Value=0
  SW_ManualControl_Lights[1Scheduler|2Manual] : Constant
  SW_TurnLights[0Off|1Left|2Right|3Both] : Constant  Value=0
  Out1 : Outport  VectorParamsAs1DForOutWhenUnconnected=off
  wires:
  SW_ManualControl_Lights[1Scheduler|2Manual]/1 -> Bus Creator1/1  "SW_ManualControl_Lights[1Scheduler|2Manual]"
  SW_TurnLights[0Off|1Left|2Right|3Both]/1 -> Bus Creator1/3  "SW_TurnLights[0Off|1Left|2Right|3Both]"
  SW_BrakeLight[0Off|1On]/1 -> Bus Creator1/2  "SW_BrakeLight[0Off|1On]"
  Bus Creator1/1 -> Out1/1

== system ASM_Traffic_new/Environment/Traffic/UserInterface/PAR_Plant/Fellow_VehicleLights/Fellow9_VehicleLights ==
  Bus Creator1 : BusCreator  Inputs=3
  SW_BrakeLight[0Off|1On] : Constant  Value=0
  SW_ManualControl_Lights[1Scheduler|2Manual] : Constant
  SW_TurnLights[0Off|1Left|2Right|3Both] : Constant  Value=0
  Out1 : Outport  VectorParamsAs1DForOutWhenUnconnected=off
  wires:
  Bus Creator1/1 -> Out1/1
  SW_BrakeLight[0Off|1On]/1 -> Bus Creator1/2  "SW_BrakeLight[0Off|1On]"
  SW_TurnLights[0Off|1Left|2Right|3Both]/1 -> Bus Creator1/3  "SW_TurnLights[0Off|1Left|2Right|3Both]"
  SW_ManualControl_Lights[1Scheduler|2Manual]/1 -> Bus Creator1/1  "SW_ManualControl_Lights[1Scheduler|2Manual]"

== system ASM_Traffic_new/VehicleDynamics/Control/SoftECU_Brake/Map_Inputs/Maneuver/S_R_FlipFlop ==
  S : Inport
  R : Inport  Port=2
  Demux : Demux  Outputs=2
      settings: DisplayOption=none
  Logic : CombinatorialLogic  TruthTable=[0 1;1 0;0 1;0 1;1 0;1 0;0 0;0 0]
  Memory : Memory  InitialCondition=initial_condition  InheritSampleTime=on
  Mux : Mux  Inputs=3
  Q : Outport  InitialOutput=0  VectorParamsAs1DForOutWhenUnconnected=off
  !Q : Outport  Port=2  InitialOutput=1  VectorParamsAs1DForOutWhenUnconnected=off
  wires:
  Demux/2 -> !Q/1
  Demux/1 -> Memory/1, Q/1
  S/1 -> Mux/1
  R/1 -> Mux/2
  Memory/1 -> Mux/3
  Mux/1 -> Logic/1
  Logic/1 -> Demux/1

== system ASM_Traffic_new/VehicleDynamics/Control/SoftECU_Brake/Map_Inputs/Maneuver/pos_edge_detection ==
  In1 : Inport
  Memory : Memory
  Relational Operator : RelationalOperator  Operator=>  OutDataTypeStr=boolean  InputSameDT=off
  Out1 : Outport  VectorParamsAs1DForOutWhenUnconnected=off
  wires:
  Memory/1 -> Relational Operator/2
  Relational Operator/1 -> Out1/1
  In1/1 -> Memory/1, Relational Operator/1

== system ASM_Traffic_new/VehicleDynamics/Control/SoftECU_Brake/Map_Inputs/Maneuver/pos_edge_detection1 ==
  In1 : Inport
  Memory : Memory
  Relational Operator : RelationalOperator  Operator=>  OutDataTypeStr=boolean  InputSameDT=off
  Out1 : Outport  VectorParamsAs1DForOutWhenUnconnected=off
  wires:
  In1/1 -> Relational Operator/1, Memory/1
  Relational Operator/1 -> Out1/1
  Memory/1 -> Relational Operator/2

== system ASM_Traffic_new/VehicleDynamics/Control/SoftECU_Brake/Map_Inputs/Maneuver/pos_edge_detection2 ==
  In1 : Inport
  Memory : Memory
  Relational Operator : RelationalOperator  Operator=>  OutDataTypeStr=boolean  InputSameDT=off
  Out1 : Outport  VectorParamsAs1DForOutWhenUnconnected=off
  wires:
  Memory/1 -> Relational Operator/2
  Relational Operator/1 -> Out1/1
  In1/1 -> Memory/1, Relational Operator/1

== system ASM_Traffic_new/VehicleDynamics/Control/SoftECU_Brake/Map_Inputs/Maneuver/pos_edge_detection3 ==
  In1 : Inport
  Memory : Memory
  Relational Operator : RelationalOperator  Operator=>  OutDataTypeStr=boolean  InputSameDT=off
  Out1 : Outport  VectorParamsAs1DForOutWhenUnconnected=off
  wires:
  In1/1 -> Relational Operator/1, Memory/1
  Relational Operator/1 -> Out1/1
  Memory/1 -> Relational Operator/2

== system ASM_Traffic_new/VehicleDynamics/Control/UserInterface/DISP_Control/ECU_Brake/Enable_p_Brake_Desired[0|1] ==
  In1 : Inport
  Out1 : Outport  VectorParamsAs1DForOutWhenUnconnected=off
  wires:
  In1/1 -> Out1/1

== system ASM_Traffic_new/VehicleDynamics/Control/UserInterface/DISP_Control/ECU_Brake/p_Brake_Desired[bar] ==
  In1 : Inport
  Out1 : Outport  VectorParamsAs1DForOutWhenUnconnected=off
  wires:
  In1/1 -> Out1/1

== system ASM_Traffic_new/VehicleDynamics/Control/UserInterface/PAR_Control/ECU_Brake/SoftECU_ESP_Switches ==
  Bus Creator : BusCreator  Inputs=3
  SW_ASR[0Off|1On] : Constant
  Sw_ESP[0Off|1ABS|2ESP] : Constant  Value=2
  Sw_ESP_Control_Mode[1ManSched|2Manual] : Constant  Value=2
  Out1 : Outport  VectorParamsAs1DForOutWhenUnconnected=off
  wires:
  Sw_ESP[0Off|1ABS|2ESP]/1 -> Bus Creator/2  "Sw_ESP[0Off|1ABS|2ESP]"
  Bus Creator/1 -> Out1/1  "ESP_Switches"
  SW_ASR[0Off|1On]/1 -> Bus Creator/3  "Sw_ASR[0Off|1On]"
  Sw_ESP_Control_Mode[1ManSched|2Manual]/1 -> Bus Creator/1  "Sw_ESP_Control_Mode[1ManSched|2Manual]"

== system ASM_Traffic_new/VehicleDynamics/Plant/UserInterface/DISP_Plant/Accelerations/a_FL_Wheel[x;y;z][m|s2] ==
  In1 : Inport
  Out1 : Outport  VectorParamsAs1DForOutWhenUnconnected=off
  wires:
  In1/1 -> Out1/1

== system ASM_Traffic_new/VehicleDynamics/Plant/UserInterface/DISP_Plant/Accelerations/a_FR_Wheel[x;y;z][m|s2] ==
  In1 : Inport
  Out1 : Outport  VectorParamsAs1DForOutWhenUnconnected=off
  wires:
  In1/1 -> Out1/1

== system ASM_Traffic_new/VehicleDynamics/Plant/UserInterface/DISP_Plant/Accelerations/a_RL_Wheel[x;y;z][m|s2] ==
  In1 : Inport
  Out1 : Outport  VectorParamsAs1DForOutWhenUnconnected=off
  wires:
  In1/1 -> Out1/1

== system ASM_Traffic_new/VehicleDynamics/Plant/UserInterface/DISP_Plant/Accelerations/a_RR_Wheel[x;y;z][m|s2] ==
  In1 : Inport
  Out1 : Outport  VectorParamsAs1DForOutWhenUnconnected=off
  wires:
  In1/1 -> Out1/1

== system ASM_Traffic_new/VehicleDynamics/Plant/UserInterface/DISP_Plant/Accelerations/a_x_Vehicle_CoG[m|s2] ==
  In1 : Inport
  Out1 : Outport  VectorParamsAs1DForOutWhenUnconnected=off
  wires:
  In1/1 -> Out1/1

== system ASM_Traffic_new/VehicleDynamics/Plant/UserInterface/DISP_Plant/Accelerations/a_y_Vehicle_CoG[m|s2] ==
  In1 : Inport
  Out1 : Outport  VectorParamsAs1DForOutWhenUnconnected=off
  wires:
  In1/1 -> Out1/1

== system ASM_Traffic_new/VehicleDynamics/Plant/UserInterface/DISP_Plant/Accelerations/a_z_Vehicle_CoG[m|s2] ==
  In1 : Inport
  Out1 : Outport  VectorParamsAs1DForOutWhenUnconnected=off
  wires:
  In1/1 -> Out1/1

== system ASM_Traffic_new/VehicleDynamics/Plant/UserInterface/DISP_Plant/Accelerations/w_Vehicle_CoG_dt[x;y;z][rad|s2] ==
  In1 : Inport
  Out1 : Outport  VectorParamsAs1DForOutWhenUnconnected=off
  wires:
  In1/1 -> Out1/1

== system ASM_Traffic_new/VehicleDynamics/Plant/UserInterface/DISP_Plant/Accelerations/w_x_Vehicle_CoG_dt[rad|s2] ==
  In1 : Inport
  Out1 : Outport  VectorParamsAs1DForOutWhenUnconnected=off
  wires:
  In1/1 -> Out1/1

== system ASM_Traffic_new/VehicleDynamics/Plant/UserInterface/DISP_Plant/Accelerations/w_y_Vehicle_CoG_dt[rad|s2] ==
  In1 : Inport
  Out1 : Outport  VectorParamsAs1DForOutWhenUnconnected=off
  wires:
  In1/1 -> Out1/1

== system ASM_Traffic_new/VehicleDynamics/Plant/UserInterface/DISP_Plant/Accelerations/w_z_Vehicle_CoG_dt[rad|s2] ==
  In1 : Inport
  Out1 : Outport  VectorParamsAs1DForOutWhenUnconnected=off
  wires:
  In1/1 -> Out1/1

== system ASM_Traffic_new/VehicleDynamics/Plant/UserInterface/DISP_Plant/Aerodynamics/F_x_Aero_CoorSys_V[N] ==
  In1 : Inport
  Out1 : Outport  VectorParamsAs1DForOutWhenUnconnected=off
  wires:
  In1/1 -> Out1/1

== system ASM_Traffic_new/VehicleDynamics/Plant/UserInterface/DISP_Plant/Aerodynamics/F_y_Aero_CoorSys_V[N] ==
  In1 : Inport
  Out1 : Outport  VectorParamsAs1DForOutWhenUnconnected=off
  wires:
  In1/1 -> Out1/1

== system ASM_Traffic_new/VehicleDynamics/Plant/UserInterface/DISP_Plant/Aerodynamics/F_z_Aero_CoorSys_V[N] ==
  In1 : Inport
  Out1 : Outport  VectorParamsAs1DForOutWhenUnconnected=off
  wires:
  In1/1 -> Out1/1

== system ASM_Traffic_new/VehicleDynamics/Plant/UserInterface/DISP_Plant/Aerodynamics/Trq_x_Aero_CoorSys_V[Nm] ==
  In1 : Inport
  Out1 : Outport  VectorParamsAs1DForOutWhenUnconnected=off
  wires:
  In1/1 -> Out1/1

== system ASM_Traffic_new/VehicleDynamics/Plant/UserInterface/DISP_Plant/Aerodynamics/Trq_y_Aero_CoorSys_V[Nm] ==
  In1 : Inport
  Out1 : Outport  VectorParamsAs1DForOutWhenUnconnected=off
  wires:
  In1/1 -> Out1/1

== system ASM_Traffic_new/VehicleDynamics/Plant/UserInterface/DISP_Plant/Aerodynamics/Trq_z_Aero_CoorSys_V[Nm] ==
  In1 : Inport
  Out1 : Outport  VectorParamsAs1DForOutWhenUnconnected=off
  wires:
  In1/1 -> Out1/1

== system ASM_Traffic_new/VehicleDynamics/Plant/UserInterface/DISP_Plant/Brake/BrakeHydraulicsModel[] ==
  In1 : Inport
  Gain : Gain
  Out1 : Outport  VectorParamsAs1DForOutWhenUnconnected=off
  wires:
  In1/1 -> Gain/1
  Gain/1 -> Out1/1

== system ASM_Traffic_new/VehicleDynamics/Plant/UserInterface/DISP_Plant/Brake/Trq_FL_Brake[Nm] ==
  In1 : Inport
  Out1 : Outport  VectorParamsAs1DForOutWhenUnconnected=off
  wires:
  In1/1 -> Out1/1

== system ASM_Traffic_new/VehicleDynamics/Plant/UserInterface/DISP_Plant/Brake/Trq_FR_Brake[Nm] ==
  In1 : Inport
  Out1 : Outport  VectorParamsAs1DForOutWhenUnconnected=off
  wires:
  In1/1 -> Out1/1

== system ASM_Traffic_new/VehicleDynamics/Plant/UserInterface/DISP_Plant/Brake/Trq_RL_Brake[Nm] ==
  In1 : Inport
  Out1 : Outport  VectorParamsAs1DForOutWhenUnconnected=off
  wires:
  In1/1 -> Out1/1

== system ASM_Traffic_new/VehicleDynamics/Plant/UserInterface/DISP_Plant/Brake/Trq_RR_Brake[Nm] ==
  In1 : Inport
  Out1 : Outport  VectorParamsAs1DForOutWhenUnconnected=off
  wires:
  In1/1 -> Out1/1

== system ASM_Traffic_new/VehicleDynamics/Plant/UserInterface/DISP_Plant/Brake/p[bar] ==
  In1 : Inport
  Out1 : Outport  VectorParamsAs1DForOutWhenUnconnected=off
  wires:
  In1/1 -> Out1/1

== system ASM_Traffic_new/VehicleDynamics/Plant/UserInterface/DISP_Plant/Brake/p_FL_Brake[bar] ==
  In1 : Inport
  Out1 : Outport  VectorParamsAs1DForOutWhenUnconnected=off
  wires:
  In1/1 -> Out1/1

== system ASM_Traffic_new/VehicleDynamics/Plant/UserInterface/DISP_Plant/Brake/p_FR_Brake[bar] ==
  In1 : Inport
  Out1 : Outport  VectorParamsAs1DForOutWhenUnconnected=off
  wires:
  In1/1 -> Out1/1

== system ASM_Traffic_new/VehicleDynamics/Plant/UserInterface/DISP_Plant/Brake/p_RL_Brake[bar] ==
  In1 : Inport
  Out1 : Outport  VectorParamsAs1DForOutWhenUnconnected=off
  wires:
  In1/1 -> Out1/1

== system ASM_Traffic_new/VehicleDynamics/Plant/UserInterface/DISP_Plant/Brake/p_RR_Brake[bar] ==
  In1 : Inport
  Out1 : Outport  VectorParamsAs1DForOutWhenUnconnected=off
  wires:
  In1/1 -> Out1/1

== system ASM_Traffic_new/VehicleDynamics/Plant/UserInterface/DISP_Plant/Brake/p_max[bar] ==
  In1 : Inport
  Out1 : Outport  VectorParamsAs1DForOutWhenUnconnected=off
  wires:
  In1/1 -> Out1/1

== system ASM_Traffic_new/VehicleDynamics/Plant/UserInterface/DISP_Plant/Overview/a_x_Vehicle_CoG[m|s2] ==
  In1 : Inport
  Out1 : Outport  VectorParamsAs1DForOutWhenUnconnected=off
  wires:
  In1/1 -> Out1/1

== system ASM_Traffic_new/VehicleDynamics/Plant/UserInterface/DISP_Plant/Overview/a_y_Vehicle_CoG[m|s2] ==
  In1 : Inport
  Out1 : Outport  VectorParamsAs1DForOutWhenUnconnected=off
  wires:
  In1/1 -> Out1/1

== system ASM_Traffic_new/VehicleDynamics/Plant/UserInterface/DISP_Plant/Overview/a_z_Vehicle_CoG[m|s2] ==
  In1 : Inport
  Out1 : Outport  VectorParamsAs1DForOutWhenUnconnected=off
  wires:
  In1/1 -> Out1/1

== system ASM_Traffic_new/VehicleDynamics/Plant/UserInterface/DISP_Plant/Overview/v_Total_Vehicle[km|h] ==
  In1 : Inport
  Out1 : Outport  VectorParamsAs1DForOutWhenUnconnected=off
  wires:
  In1/1 -> Out1/1

== system ASM_Traffic_new/VehicleDynamics/Plant/UserInterface/DISP_Plant/Overview/v_x_Vehicle_CoG[km|h] ==
  In1 : Inport
  Out1 : Outport  VectorParamsAs1DForOutWhenUnconnected=off
  wires:
  In1/1 -> Out1/1

== system ASM_Traffic_new/VehicleDynamics/Plant/UserInterface/DISP_Plant/Overview/v_y_Vehicle_CoG[km|h] ==
  In1 : Inport
  Out1 : Outport  VectorParamsAs1DForOutWhenUnconnected=off
  wires:
  In1/1 -> Out1/1

== system ASM_Traffic_new/VehicleDynamics/Plant/UserInterface/DISP_Plant/Overview/v_z_Vehicle_CoG[km|h] ==
  In1 : Inport
  Out1 : Outport  VectorParamsAs1DForOutWhenUnconnected=off
  wires:
  In1/1 -> Out1/1

== system ASM_Traffic_new/VehicleDynamics/Plant/UserInterface/DISP_Plant/Positions/Angle_Pitch_Vehicle_CoorSys_E[deg] ==
  In1 : Inport
  Out1 : Outport  VectorParamsAs1DForOutWhenUnconnected=off
  wires:
  In1/1 -> Out1/1

== system ASM_Traffic_new/VehicleDynamics/Plant/UserInterface/DISP_Plant/Positions/Angle_Roll_Vehicle_CoorSys_E[deg] ==
  In1 : Inport
  Out1 : Outport  VectorParamsAs1DForOutWhenUnconnected=off
  wires:
  In1/1 -> Out1/1

== system ASM_Traffic_new/VehicleDynamics/Plant/UserInterface/DISP_Plant/Positions/Angle_Yaw_Vehicle_CoorSys_E[deg] ==
  In1 : Inport
  Out1 : Outport  VectorParamsAs1DForOutWhenUnconnected=off
  wires:
  In1/1 -> Out1/1

== system ASM_Traffic_new/VehicleDynamics/Plant/UserInterface/DISP_Plant/Positions/Pos_x_Vehicle_CoorSys_E[m] ==
  In1 : Inport
  Out1 : Outport  VectorParamsAs1DForOutWhenUnconnected=off
  wires:
  In1/1 -> Out1/1

== system ASM_Traffic_new/VehicleDynamics/Plant/UserInterface/DISP_Plant/Positions/Pos_y_Vehicle_CoorSys_E[m] ==
  In1 : Inport
  Out1 : Outport  VectorParamsAs1DForOutWhenUnconnected=off
  wires:
  In1/1 -> Out1/1

== system ASM_Traffic_new/VehicleDynamics/Plant/UserInterface/DISP_Plant/Positions/Pos_z_Vehicle_CoorSys_E[m] ==
  In1 : Inport
  Out1 : Outport  VectorParamsAs1DForOutWhenUnconnected=off
  wires:
  In1/1 -> Out1/1

== system ASM_Traffic_new/VehicleDynamics/Plant/UserInterface/DISP_Plant/Positions/s_Vehicle[m] ==
  In1 : Inport
  Out1 : Outport  VectorParamsAs1DForOutWhenUnconnected=off
  wires:
  In1/1 -> Out1/1

== system ASM_Traffic_new/VehicleDynamics/Plant/UserInterface/DISP_Plant/Sensor1/a_Angular_Sensor1_CoorSys_VH[x;y;z][rad|s2] ==
  In1 : Inport
  Out1 : Outport  VectorParamsAs1DForOutWhenUnconnected=off
  wires:
  In1/1 -> Out1/1

== system ASM_Traffic_new/VehicleDynamics/Plant/UserInterface/DISP_Plant/Sensor1/a_Angular_Sensor1_CoorSys_V[x;y;z][rad|s2] ==
  In1 : Inport
  Out1 : Outport  VectorParamsAs1DForOutWhenUnconnected=off
  wires:
  In1/1 -> Out1/1
